simulink model "afe_inv_psm_param"  (R2026b)
settings: Solver=ode23t  StopTime=param.sim.simlength  FixedStep=tc  MaxStep=param.glb_time.tc  RelTol=1e-4
values from neighbouring files (symbols this model uses):
  param = add_template_extras(param, options)    [init_model.m]
undefined symbols (not defined in the file or in its folder): magnitude, omega_m_bez
libraries: fl_lib x330, nesl_utility x174, igbt_simple_2th_lib x12, moving_average_filter x10, moving_average_filter_cc x8, sl_discontinuities x3, single_phase_transformer_lib x3, linear_double_integrator_observer_ccaller x2, discrete_time_low_pass_filter x2, threephase_inductor_lib x2, three_phase_pwm_modulator x2, three_phase_inverter_ideal_switch_based_model x2
(part 2 of 13)

== system afe_inv_psm_param/grid/power meter iec mfunc ==
  Bus Selector : BusSelector  OutputSignals=Q1p,Q1n,P1n,P1p,U1n,U1p,i_act_1n,i_react_1n,i_act_1p,i_react_1p
  Constant : Constant  Value=param.glb_time.ts_afe
  Step : Step  Time=0.025  InitialValue=1  FinalValue=0  SampleTime=0
  To Workspace1 : ToWorkspace  VariableName=i_react_1n  SampleTime=param.glb_time.ts_afe
      settings: MaxDataPoints=param.glb_time.Ns_afe
  To Workspace2 : ToWorkspace  VariableName=i_react_1p  SampleTime=param.glb_time.ts_afe
      settings: MaxDataPoints=param.glb_time.Ns_afe
  To Workspace3 : ToWorkspace  VariableName=i_act_1n  SampleTime=param.glb_time.ts_afe
      settings: MaxDataPoints=param.glb_time.Ns_afe
  To Workspace4 : ToWorkspace  VariableName=i_act_1p  SampleTime=param.glb_time.ts_afe
      settings: MaxDataPoints=param.glb_time.Ns_afe
  To Workspace5 : ToWorkspace  VariableName=u1p  SampleTime=param.glb_time.ts_afe
      settings: MaxDataPoints=param.glb_time.Ns_afe
  To Workspace6 : ToWorkspace  VariableName=u1n  SampleTime=param.glb_time.ts_afe
      settings: MaxDataPoints=param.glb_time.Ns_afe
  Zero-Order Hold{,1..5} (6 alike) : ZeroOrderHold  SampleTime=param.glb_time.ts_afe
  three_phase_power_meter_iec : MATLAB Function  TreatAsAtomicUnit=on  SystemSampleTime=param.glb_time.ts_afe
  tag scope: P1n_global=global, P1p_global=global, Q1n_global=global, Q1p_global=global
  wires:
  Bus Selector/6 -> To Workspace5/1  "<U1p>"
  Bus Selector/8 -> To Workspace1/1  "<i_react_1n>"
  Bus Selector/10 -> To Workspace2/1  "<i_react_1p>"
  Bus Selector/5 -> To Workspace6/1  "<U1n>"
  Bus Selector/4 -> [P1p_global]  "<P1p>"
  Bus Selector/2 -> [Q1n_global]  "<Q1n>"
  Bus Selector/1 -> [Q1p_global]  "<Q1p>"
  Bus Selector/7 -> To Workspace3/1  "<i_act_1n>"
  Bus Selector/9 -> To Workspace4/1  "<i_act_1p>"
  Bus Selector/3 -> [P1n_global]  "<P1n>"
  three_phase_power_meter_iec/1(m) -> Bus Selector/1
  Zero-Order Hold/1 -> three_phase_power_meter_iec/1(phase)
  Zero-Order Hold2/1 -> three_phase_power_meter_iec/3(i_abc)
  [phase_grid_emulator] -> Zero-Order Hold/1
  Step/1 -> Zero-Order Hold5/1
  Zero-Order Hold3/1 -> three_phase_power_meter_iec/4(omega)
  Zero-Order Hold4/1 -> three_phase_power_meter_iec/5(ts)
  [ug_abc] -> Zero-Order Hold1/1
  Zero-Order Hold5/1 -> three_phase_power_meter_iec/6(enable_time)
  [ig_abc] -> Zero-Order Hold2/1
  [omega_grid_emulator] -> Zero-Order Hold3/1
  Constant/1 -> Zero-Order Hold4/1
  Zero-Order Hold1/1 -> three_phase_power_meter_iec/2(u_abc)

== system afe_inv_psm_param/grid/threephase_vi_measures ==
  Bus Creator : BusCreator  Inputs=6
  Current Sensor : fl_lib/Electrical/Electrical Sensors/Current Sensor
  Current Sensor1 : fl_lib/Electrical/Electrical Sensors/Current Sensor
  Current Sensor2 : fl_lib/Electrical/Electrical Sensors/Current Sensor
  Electrical Reference1 : fl_lib/Electrical/Electrical Elements/Electrical Reference
  Selector : Selector  InputPortWidth=6  IndexOptions=Index vector (dialog)  Indices=[1 2 3]  OutputSizes=1  RuntimeRangeChecks=off
  Selector1 : Selector  InputPortWidth=6  IndexOptions=Index vector (dialog)  Indices=[4 5 6]  OutputSizes=1  RuntimeRangeChecks=off
  Voltage Sensor : fl_lib/Electrical/Electrical Sensors/Voltage Sensor
  Voltage Sensor1 : fl_lib/Electrical/Electrical Sensors/Voltage Sensor
  Voltage Sensor2 : fl_lib/Electrical/Electrical Sensors/Voltage Sensor
  ia_grid : nesl_utility/PS-Simulink Converter  PhysicalDomain=network_engine_domain  SubClassName=ps_output  LeftPortType=input  RightPortType=output  PseudoPeriodic=off  Frequencies=[]  VectorFormat=1-D array  Unit=A  AffineConversion=off
  ib_grid : nesl_utility/PS-Simulink Converter  PhysicalDomain=network_engine_domain  SubClassName=ps_output  LeftPortType=input  RightPortType=output  PseudoPeriodic=off  Frequencies=[]  VectorFormat=1-D array  Unit=A  AffineConversion=off
  ic_grid : nesl_utility/PS-Simulink Converter  PhysicalDomain=network_engine_domain  SubClassName=ps_output  LeftPortType=input  RightPortType=output  PseudoPeriodic=off  Frequencies=[]  VectorFormat=1-D array  Unit=A  AffineConversion=off
  ig_abc/ug_abc : Scope  NumInputPorts=2
      settings: SampleTime=param.glb_time.tc  ActiveDisplayYMinimum=-728.92703752654245  ActiveDisplayYMaximum=734.90808013997  DataLoggingVariableName=ScopeData2
  ua_grid : nesl_utility/PS-Simulink Converter  PhysicalDomain=network_engine_domain  SubClassName=ps_output  LeftPortType=input  RightPortType=output  PseudoPeriodic=off  Frequencies=[]  VectorFormat=1-D array  Unit=V  AffineConversion=off
  ub_grid : nesl_utility/PS-Simulink Converter  PhysicalDomain=network_engine_domain  SubClassName=ps_output  LeftPortType=input  RightPortType=output  PseudoPeriodic=off  Frequencies=[]  VectorFormat=1-D array  Unit=V  AffineConversion=off
  uc_grid : nesl_utility/PS-Simulink Converter  PhysicalDomain=network_engine_domain  SubClassName=ps_output  LeftPortType=input  RightPortType=output  PseudoPeriodic=off  Frequencies=[]  VectorFormat=1-D array  Unit=V  AffineConversion=off
  Ua : PMIOPort  Side=Left
  ua : PMIOPort  Port=2  Side=Right
  Ub : PMIOPort  Port=3  Side=Left
  ub : PMIOPort  Port=4  Side=Right
  Uc : PMIOPort  Port=5  Side=Left
  uc : PMIOPort  Port=6  Side=Right
  tag scope: ig_abc=global, ug_abc=global
  wires:
  Bus Creator/1 -> Selector1/1, Selector/1  "vi_data"
  Selector/1 -> [ug_abc]
  ib_grid/1 -> Bus Creator/5  "ib"
  ia_grid/1 -> Bus Creator/4  "ia"
  ic_grid/1 -> Bus Creator/6  "ic"
  ua_grid/1 -> Bus Creator/1  "ua"
  ub_grid/1 -> Bus Creator/2  "ub"
  uc_grid/1 -> Bus Creator/3  "uc"
  Selector1/1 -> [ig_abc]
  [ug_abc] -> ig_abc/ug_abc/2  "ug_abc(line)"
  [ig_abc] -> ig_abc/ug_abc/1  "ig_abc(line)"
  connections:
  Current Sensor1/LConn1 -- Ub/RConn1 -- Voltage Sensor1/LConn1
  Electrical Reference1/LConn1 -- Voltage Sensor/RConn2 -- Voltage Sensor2/RConn2 -- Voltage Sensor1/RConn2
  Voltage Sensor/RConn1 -- ua_grid/LConn1
  Current Sensor/RConn2 -- ua/RConn1
  Voltage Sensor1/RConn1 -- ub_grid/LConn1
  Voltage Sensor2/LConn1 -- Current Sensor2/LConn1 -- Uc/RConn1
  Current Sensor/LConn1 -- Ua/RConn1 -- Voltage Sensor/LConn1
  Current Sensor1/RConn2 -- ub/RConn1
  Voltage Sensor2/RConn1 -- uc_grid/LConn1
  ib_grid/LConn1 -- Current Sensor1/RConn1
  ia_grid/LConn1 -- Current Sensor/RConn1
  ic_grid/LConn1 -- Current Sensor2/RConn1
  Current Sensor2/RConn2 -- uc/RConn1

== system afe_inv_psm_param/inverter_measurement_sim/igbt_power_losses ==
  To Workspace12 : ToWorkspace  VariableName=igbt_ploss_invQ1_sim  SampleTime=param.glb_time.tc
      settings: MaxDataPoints=param.glb_time.Nc
  To Workspace14 : ToWorkspace  VariableName=igbt_current_invQ1_sim  SampleTime=param.glb_time.tc
      settings: MaxDataPoints=param.glb_time.Nc
  To Workspace15 : ToWorkspace  VariableName=igbt_voltage_invQ1_sim  SampleTime=param.glb_time.tc
      settings: MaxDataPoints=param.glb_time.Nc
  To Workspace16 : ToWorkspace  VariableName=igbt_JH_temp_invQ1_sim  SampleTime=param.glb_time.tc
      settings: MaxDataPoints=param.glb_time.Nc
  To Workspace17 : ToWorkspace  VariableName=igbt_HA_temp_invQ1_sim  SampleTime=param.glb_time.tc
      settings: MaxDataPoints=param.glb_time.Nc
  To Workspace18 : ToWorkspace  VariableName=diode_ploss_invQ1_sim  SampleTime=param.glb_time.tc
      settings: MaxDataPoints=param.glb_time.Nc
  To Workspace19 : ToWorkspace  VariableName=diode_JH_temp_invQ1_sim  SampleTime=param.glb_time.tc
      settings: MaxDataPoints=param.glb_time.Nc
  To Workspace20 : ToWorkspace  VariableName=diode_HA_temp_invQ1_sim  SampleTime=param.glb_time.tc
      settings: MaxDataPoints=param.glb_time.Nc
  wires:
  [igbt_ploss_invQ1] -> To Workspace12/1  "igbt_ploss_invQ1"
  [igbt_current_invQ1] -> To Workspace14/1  "igbt_current_invQ1"
  [igbt_voltage_invQ1] -> To Workspace15/1  "igbt_voltage_invQ1"
  [diode_JH_temp_invQ1] -> To Workspace19/1  "diode_JH_temp_invQ1"
  [igbt_JH_temp_invQ1] -> To Workspace16/1  "igbt_JH_temp_invQ1"
  [diode_HA_temp_invQ1] -> To Workspace20/1  "diode_HA_temp_invQ1"
  [igbt_HA_temp_invQ1] -> To Workspace17/1  "igbt_HA_temp_invQ1"
  [diode_ploss_invQ1] -> To Workspace18/1  "diode_ploss_invQ1"

== system afe_inv_psm_param/inverter_measurement_sim/module_1 ==
  To Workspace12 : ToWorkspace  VariableName=ileg_dc_inv_sim_mod1  SampleTime=param.glb_time.tc
      settings: MaxDataPoints=param.glb_time.Nc
  To Workspace14 : ToWorkspace  VariableName=is_uvw_sim_mod1  SampleTime=param.glb_time.tc
      settings: MaxDataPoints=param.glb_time.Nc
  To Workspace15 : ToWorkspace  VariableName=us_uvw_sim_mod1  SampleTime=param.glb_time.tc
      settings: MaxDataPoints=param.glb_time.Nc
  wires:
  [us_uvw_pu_mod1] -> To Workspace15/1
  [ileg_dc_inv_mod1] -> To Workspace12/1
  [is_uvw_pu_mod1] -> To Workspace14/1

== system afe_inv_psm_param/pmsm/synchronous_motor ==
  Bus Selector : BusSelector  OutputSignals=psi_r_alpha (Vs)
  Bus Selector1 : BusSelector  OutputSignals=psi_r_alpha (Vs)
  Bus Selector10 : BusSelector  OutputSignals=uq (V)
  Bus Selector11 : BusSelector  OutputSignals=ud (V)
  Bus Selector12 : BusSelector  OutputSignals=iq (A)
  Bus Selector13 : BusSelector  OutputSignals=id (A)
  Bus Selector2 : BusSelector  OutputSignals=iu (A)
  Bus Selector3 : BusSelector  OutputSignals=iv (A)
  Bus Selector4 : BusSelector  OutputSignals=iw (A)
  Bus Selector5 : BusSelector  OutputSignals=omega_elec (rad/s)
  Bus Selector6 : BusSelector  OutputSignals=phase_elec (rad)
  Bus Selector7 : BusSelector  OutputSignals=pwr_in (kW)
  Bus Selector8 : BusSelector  OutputSignals=pwr_out (kW)
  Bus Selector9 : BusSelector  OutputSignals=torque (Nm)
  Open Circuit : fl_lib/Electrical/Electrical Elements/Open Circuit  v_specify=off  v_priority=None  v=0 V  v_nominal_specify=off  v_nominal_value=1  v_nominal_unit=V
  permanent_magnet_synchronous_machine : permanent_magnet_synchronous_machine/permanent_magnet_synchronous_machine  pp=param.psm.machine.number_poles  psi_m=param.psm.machine.psi_m  Lmu=param.psm.machine.Lmu  La=param.psm.machine.La_m  Lb=param.psm.machine.Lb_m  Rs=param.psm.machine.Rs_m  Jm=param.psm.machine.Jm_m  b_linear=param.psm.machine.load_friction_m  b_quadratic=0  h5_percent=0  h7_percent=0  psi_r_u_init=param.psm.machine.psi_m  psi_r_v_init=-param.psm.machine.psi_m/2  psi_r_w_init=-param.psm.machine.psi_m/2  omega_init=0  phase_init=0  angle_error=0
  shaft : PMIOPort  Side=Right
  u : PMIOPort  Port=2  Side=Left
  v : PMIOPort  Port=3  Side=Left
  w : PMIOPort  Port=4  Side=Left
  psi_m : PMIOPort  Port=5  Side=Left
  motor_data : Outport
  tag scope: id_psm=global, iq_psm=global, iu_psm=global, iv_psm=global, iw_psm=global, omega_elec_psm=global, psi_r_alpha_psm=global, psi_r_beta_psm=global, pwr_in_psm=global, pwr_out_psm=global, theta_elec_psm=global, torque_load_psm=global, ud_psm=global, uq_psm=global
  wires:
  permanent_magnet_synchronous_machine/1 -> Bus Selector8/1, Bus Selector10/1, Bus Selector11/1, Bus Selector12/1, Bus Selector13/1, Bus Selector9/1, Bus Selector7/1, Bus Selector6/1, Bus Selector5/1, Bus Selector4/1, Bus Selector3/1, Bus Selector2/1, Bus Selector1/1, Bus Selector/1, motor_data/1
  Bus Selector/1 -> [psi_r_alpha_psm]  "<psi_r_alpha (Vs)>"
  Bus Selector1/1 -> [psi_r_beta_psm]  "<psi_r_alpha (Vs)>"
  Bus Selector2/1 -> [iu_psm]  "<iu (A)>"
  Bus Selector3/1 -> [iv_psm]  "<iv (A)>"
  Bus Selector4/1 -> [iw_psm]  "<iw (A)>"
  Bus Selector5/1 -> [omega_elec_psm]  "<omega_elec (rad/s)>"
  Bus Selector6/1 -> [theta_elec_psm]  "<phase_elec (rad)>"
  Bus Selector7/1 -> [pwr_in_psm]  "<pwr_in (kW)>"
  Bus Selector8/1 -> [pwr_out_psm]  "<pwr_out (kW)>"
  Bus Selector9/1 -> [torque_load_psm]  "<torque (Nm)>"
  Bus Selector10/1 -> [uq_psm]  "<uq (V)>"
  Bus Selector11/1 -> [ud_psm]  "<ud (V)>"
  Bus Selector12/1 -> [iq_psm]  "<iq (A)>"
  Bus Selector13/1 -> [id_psm]  "<id (A)>"
  connections:
  permanent_magnet_synchronous_machine/RConn1 -- shaft/RConn1
  permanent_magnet_synchronous_machine/LConn1 -- u/RConn1
  permanent_magnet_synchronous_machine/LConn2 -- v/RConn1
  permanent_magnet_synchronous_machine/LConn3 -- w/RConn1
  permanent_magnet_synchronous_machine/LConn4 -- psi_m/RConn1
  permanent_magnet_synchronous_machine/LConn5 -- Open Circuit/LConn1

== system afe_inv_psm_param/scopes/cable_effects ==
  cable_effects : Scope  NumInputPorts=3
      settings: SampleTime=param.glb_time.tc  ActiveDisplayYMinimum=-7.1054273576010019E-14  ActiveDisplayYMaximum=7.1054273576010019E-14  DataLoggingVariableName=ScopeData35
  wires:
  [udc_pgnd] -> cable_effects/2
  [udc_ngnd] -> cable_effects/3
  [is_uvw_cm_mod1] -> cable_effects/1

== system afe_inv_psm_param/scopes/grid_afe_side ==
  Gain7 : Gain  Gain=param.afe.hw.ibez
  Gain8 : Gain  Gain=param.afe.hw.ubez
  Gain9 : Gain  Gain=param.afe.hw.ibez
  IEC_power_meter : Scope  NumInputPorts=4
      settings: ActiveDisplayYMinimum=-221704.59704037459  ActiveDisplayYMaximum=262876.57731367293  DataLoggingVariableName=ScopeData14
  i_line_abc/u_line_abc : Scope  NumInputPorts=2
      settings: SampleTime=param.glb_time.tc  ActiveDisplayYMinimum=-1352.5734119476883  ActiveDisplayYMaximum=1505.395019752161  DataLoggingVariableName=ScopeData20
  idc/udc : Scope  NumInputPorts=2
      settings: SampleTime=param.glb_time.tc  ActiveDisplayYMinimum=-237.45231016815259  ActiveDisplayYMaximum=320.54398715417091  DataLoggingVariableName=ScopeData23
  ig_abc/ug_abc _mod1 : Scope  NumInputPorts=2
      settings: SampleTime=param.glb_time.tc  ActiveDisplayYMinimum=-4.4957016262667837  ActiveDisplayYMaximum=4.3239423057982735  DataLoggingVariableName=ScopeData22
  is_abc/us_abc _mod1 : Scope  NumInputPorts=3
      settings: SampleTime=param.glb_time.tc  ActiveDisplayYMinimum=-2620.8441075302808  ActiveDisplayYMaximum=2310.3545900694107  DataLoggingVariableName=ScopeData21
  udc voltages : Scope  NumInputPorts=2
      settings: SampleTime=param.glb_time.tc  ActiveDisplayYMinimum=-0.1691941690232826  ActiveDisplayYMaximum=1.5064339432334795  DataLoggingVariableName=ScopeData24
  wires:
  [udc_mod1] -> idc/udc/2  "udc_dclink_mod1"
  [ug_abc_pu_mod1] -> ig_abc/ug_abc _mod1/2  "ug_abc_mod1"
  Gain8/1 -> is_abc/us_abc _mod1/2  "vs_abc_mod1"
  [ic_dclink_mod1] -> idc/udc/1  "ic_dclink_mod1"
  [is_abc_pu_mod1] -> Gain7/1
  [Q1p_global] -> IEC_power_meter/2  "Q1p_global"
  [all_voltages_about_dclink] -> udc voltages/2  "all_voltages_about_dclink"
  Gain7/1 -> is_abc/us_abc _mod1/1  "is_abc_mod1"
  [iz_afe_pu_mod1] -> Gain9/1
  [i_abc_line] -> i_line_abc/u_line_abc/1  "i_abc_line"
  [u_abc_line] -> i_line_abc/u_line_abc/2  "u_abc_line"
  [P1n_global] -> IEC_power_meter/4  "P1n_global"
  [ig_abc_pu_mod1] -> ig_abc/ug_abc _mod1/1  "ig_abc_mod1"
  [vs_abc_pu_mod1] -> Gain8/1
  [vdc_pu_afe_mod1] -> udc voltages/1  "udc"
  Gain9/1 -> is_abc/us_abc _mod1/3  "iz_afe_mod1"
  [Q1n_global] -> IEC_power_meter/1  "Q1n_global"
  [P1p_global] -> IEC_power_meter/3  "P1p_global"

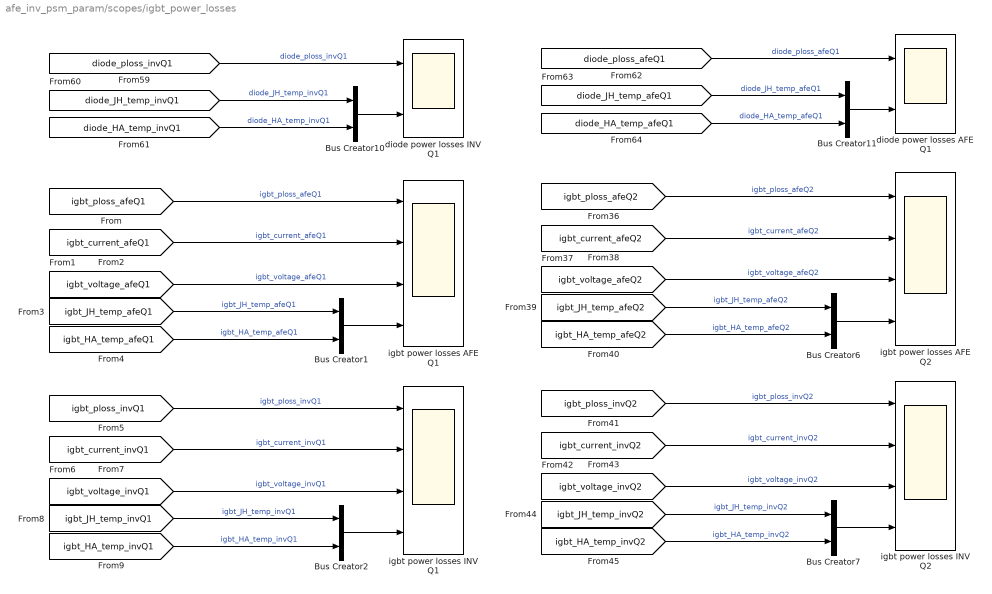
== system afe_inv_psm_param/scopes/igbt_power_losses ==
  Bus Creator{1..2,6..7,10..11} (6 alike) : BusCreator  Inputs=2
  diode power losses AFE Q1 : Scope  NumInputPorts=2
      settings: SampleTime=param.glb_time.tc  ActiveDisplayYMinimum=-0.87039317174009745  ActiveDisplayYMaximum=7.8312553964690395  DataLoggingVariableName=ScopeData32
  diode power losses INV Q1 : Scope  NumInputPorts=2
      settings: SampleTime=param.glb_time.tc  ActiveDisplayYMinimum=-1  ActiveDisplayYMaximum=1  DataLoggingVariableName=ScopeData31
  igbt power losses AFE Q1 : Scope  NumInputPorts=4
      settings: SampleTime=param.glb_time.tc  ActiveDisplayYMinimum=-49.038943467813  ActiveDisplayYMaximum=441.3504912103171  DataLoggingVariableName=ScopeData15
  igbt power losses AFE Q2 : Scope  NumInputPorts=4
      settings: SampleTime=param.glb_time.tc  ActiveDisplayYMinimum=-40.410135398015626  ActiveDisplayYMaximum=363.69121858214072  DataLoggingVariableName=ScopeData26
  igbt power losses INV Q1 : Scope  NumInputPorts=4
      settings: SampleTime=param.glb_time.tc  ActiveDisplayYMinimum=-36.37444736851036  ActiveDisplayYMaximum=327.37002631659328  DataLoggingVariableName=ScopeData16
  igbt power losses INV Q2 : Scope  NumInputPorts=4
      settings: SampleTime=param.glb_time.tc  ActiveDisplayYMinimum=-6409.6577502266955  ActiveDisplayYMaximum=762.94403267363941  DataLoggingVariableName=ScopeData27
  wires:
  [igbt_ploss_afeQ1] -> igbt power losses AFE Q1/1  "igbt_ploss_afeQ1"
  [igbt_JH_temp_invQ1] -> Bus Creator2/1  "igbt_JH_temp_invQ1"
  [diode_JH_temp_invQ1] -> Bus Creator10/1  "diode_JH_temp_invQ1"
  [igbt_HA_temp_invQ2] -> Bus Creator7/2  "igbt_HA_temp_invQ2"
  [igbt_current_afeQ2] -> igbt power losses AFE Q2/2  "igbt_current_afeQ2"
  [igbt_ploss_afeQ2] -> igbt power losses AFE Q2/1  "igbt_ploss_afeQ2"
  [igbt_current_invQ1] -> igbt power losses INV Q1/2  "igbt_current_invQ1"
  [igbt_JH_temp_afeQ1] -> Bus Creator1/1  "igbt_JH_temp_afeQ1"
  [igbt_current_invQ2] -> igbt power losses INV Q2/2  "igbt_current_invQ2"
  [diode_JH_temp_afeQ1] -> Bus Creator11/1  "diode_JH_temp_afeQ1"
  [igbt_HA_temp_invQ1] -> Bus Creator2/2  "igbt_HA_temp_invQ1"
  [igbt_JH_temp_afeQ2] -> Bus Creator6/1  "igbt_JH_temp_afeQ2"
  Bus Creator11/1 -> diode power losses AFE Q1/2
  [diode_ploss_invQ1] -> diode power losses INV Q1/1  "diode_ploss_invQ1"
  [igbt_ploss_invQ1] -> igbt power losses INV Q1/1  "igbt_ploss_invQ1"
  [igbt_HA_temp_afeQ2] -> Bus Creator6/2  "igbt_HA_temp_afeQ2"
  Bus Creator7/1 -> igbt power losses INV Q2/4
  [igbt_voltage_invQ2] -> igbt power losses INV Q2/3  "igbt_voltage_invQ2"
  Bus Creator10/1 -> diode power losses INV Q1/2
  [igbt_JH_temp_invQ2] -> Bus Creator7/1  "igbt_JH_temp_invQ2"
  [diode_HA_temp_afeQ1] -> Bus Creator11/2  "diode_HA_temp_afeQ1"
  Bus Creator1/1 -> igbt power losses AFE Q1/4
  Bus Creator6/1 -> igbt power losses AFE Q2/4
  [igbt_voltage_afeQ1] -> igbt power losses AFE Q1/3  "igbt_voltage_afeQ1"
  [igbt_current_afeQ1] -> igbt power losses AFE Q1/2  "igbt_current_afeQ1"
  [igbt_HA_temp_afeQ1] -> Bus Creator1/2  "igbt_HA_temp_afeQ1"
  [diode_ploss_afeQ1] -> diode power losses AFE Q1/1  "diode_ploss_afeQ1"
  Bus Creator2/1 -> igbt power losses INV Q1/4
  [diode_HA_temp_invQ1] -> Bus Creator10/2  "diode_HA_temp_invQ1"
  [igbt_voltage_invQ1] -> igbt power losses INV Q1/3  "igbt_voltage_invQ1"
  [igbt_ploss_invQ2] -> igbt power losses INV Q2/1  "igbt_ploss_invQ2"
  [igbt_voltage_afeQ2] -> igbt power losses AFE Q2/3  "igbt_voltage_afeQ2"

== system afe_inv_psm_param/scopes/machine_side ==
  Bus Creator3 : BusCreator  Inputs=2
  Bus Creator4 : BusCreator  Inputs=2
  Bus Creator5 : BusCreator  Inputs=2
  From56 : From  Commented=on  GotoTag=inverter_voltage_ee_phase_u
  From57 : From  Commented=on  GotoTag=inverter_voltage_ee_phase_v
  From58 : From  Commented=on  GotoTag=inverter_voltage_ee_phase_w
  Gain1 : Gain  Gain=1e-3
  LTI System : cstblocks_lti/LTI System  sys=param.ctrl.filters.inv.SOF_50Hz.ss_c  IC=[]  PadeOrder=0
  LTI System1 : cstblocks_lti/LTI System  sys=param.ctrl.filters.inv.SOF_50Hz.ss_c  IC=[]  PadeOrder=0
  inverter_voltage_ee : Scope  Commented=on  NumInputPorts=3
      settings: SampleTime=param.sim.tc  ActiveDisplayYMinimum=-207.5782073641667  ActiveDisplayYMaximum=1301.7632755987056  DataLoggingVariableName=ScopeData30
  is_uvw/us_uvw : Scope  NumInputPorts=2
      settings: SampleTime=param.glb_time.tc  ActiveDisplayYMinimum=-1.2325569675038333  ActiveDisplayYMaximum=1.2339333833020862  DataLoggingVariableName=ScopeData25
  motor currents : Scope  NumInputPorts=3
      settings: SampleTime=param.glb_time.tc  ActiveDisplayYMinimum=-232.58671124644178  ActiveDisplayYMaximum=232.76282128626991  DataLoggingVariableName=ScopeData17
  motor dq : Scope  NumInputPorts=2
      settings: SampleTime=param.glb_time.tc  ActiveDisplayYMinimum=-850.02239826316088  ActiveDisplayYMaximum=207.16586596148719  DataLoggingVariableName=ScopeData18
  motor mech : Scope  NumInputPorts=3
      settings: SampleTime=param.glb_time.tc  ActiveDisplayYMinimum=-2.216582738378952  ActiveDisplayYMaximum=19.949244645410573  DataLoggingVariableName=ScopeData11
  phi_alpha_pmsm/phi_beta_pmsm : Scope  NumInputPorts=2
      settings: SampleTime=param.glb_time.tc  ActiveDisplayYMinimum=-4.8008048511588592  ActiveDisplayYMaximum=4.8008564448893649  DataLoggingVariableName=ScopeData19
  wires:
  [iu_psm] -> motor currents/1  "iu_psm"
  [psi_r_beta_psm] -> phi_alpha_pmsm/phi_beta_pmsm/2
  [id_psm] -> Bus Creator4/2  "id_psm"
  [ud_psm] -> Bus Creator3/1  "ud_psm"
  Bus Creator4/1 -> motor dq/2
  [iq_psm] -> Bus Creator4/1  "iq_psm"
  [uq_psm] -> Bus Creator3/2  "uq_psm"
  Bus Creator3/1 -> motor dq/1
  [psi_r_alpha_psm] -> phi_alpha_pmsm/phi_beta_pmsm/1
  [iv_psm] -> motor currents/2  "iv_psm"
  [iw_psm] -> motor currents/3  "iw_psm"
  [pwr_in_psm] -> LTI System/1
  LTI System1/1 -> Bus Creator5/2  "pwr_out_psm (kW)"
  [torque_load_psm] -> Gain1/1
  LTI System/1 -> Bus Creator5/1  "pin_psm (kW)"
  Gain1/1 -> motor mech/2  "torque_load_psm (kNm)"
  [rpm_motor] -> motor mech/1  "omega_elec_psm (rpm)"
  Bus Creator5/1 -> motor mech/3
  [pwr_out_psm] -> LTI System1/1
  [us_uvw_pu_mod1] -> is_uvw/us_uvw/2  "us_uvw_pu_mod1"
  [is_uvw_pu_mod1] -> is_uvw/us_uvw/1  "is_uvw_pu_mod1"
  From58/1 -> inverter_voltage_ee/3  "inverter_voltage_ee_phase_w"
  From56/1 -> inverter_voltage_ee/1  "inverter_voltage_ee_phase_u"
  From57/1 -> inverter_voltage_ee/2  "inverter_voltage_ee_phase_v"

== system afe_inv_psm_param/scopes/mosfet_power_losses ==
  Bus Creator8 : BusCreator  Inputs=2
  Bus Creator9 : BusCreator  Inputs=2
  mosfet power losses INV Q1 : Scope  NumInputPorts=4
      settings: SampleTime=param.glb_time.tc  ActiveDisplayYMinimum=-52.647210306071649  ActiveDisplayYMaximum=473.81757031333393  DataLoggingVariableName=ScopeData28
  mosfet power losses INV Q2 : Scope  NumInputPorts=4
      settings: SampleTime=param.glb_time.tc  ActiveDisplayYMinimum=-60.051099059926763  ActiveDisplayYMaximum=540.45256909803  DataLoggingVariableName=ScopeData29
  wires:
  [mosfet_current_invQ2] -> mosfet power losses INV Q2/3  "mosfet_current_invQ2"
  [mosfet_voltage_invQ1] -> mosfet power losses INV Q1/2  "mosfet_voltage_invQ1"
  [mosfet_HA_temp_invQ2] -> Bus Creator9/2  "mosfet_HA_temp_invQ2"
  [mosfet_JH_temp_invQ2] -> Bus Creator9/1  "mosfet_JH_temp_invQ2"
  [mosfet_ploss_invQ1] -> mosfet power losses INV Q1/1  "mosfet_ploss_invQ1"
  [mosfet_HA_temp_invQ1] -> Bus Creator8/2  "mosfet_HA_temp_invQ1"
  [mosfet_current_invQ1] -> mosfet power losses INV Q1/3  "mosfet_current_invQ1"
  Bus Creator8/1 -> mosfet power losses INV Q1/4
  [mosfet_voltage_invQ2] -> mosfet power losses INV Q2/2  "mosfet_voltage_invQ2"
  [mosfet_ploss_invQ2] -> mosfet power losses INV Q2/1  "mosfet_ploss_invQ2"
  Bus Creator9/1 -> mosfet power losses INV Q2/4
  [mosfet_JH_temp_invQ1] -> Bus Creator8/1  "mosfet_JH_temp_invQ1"

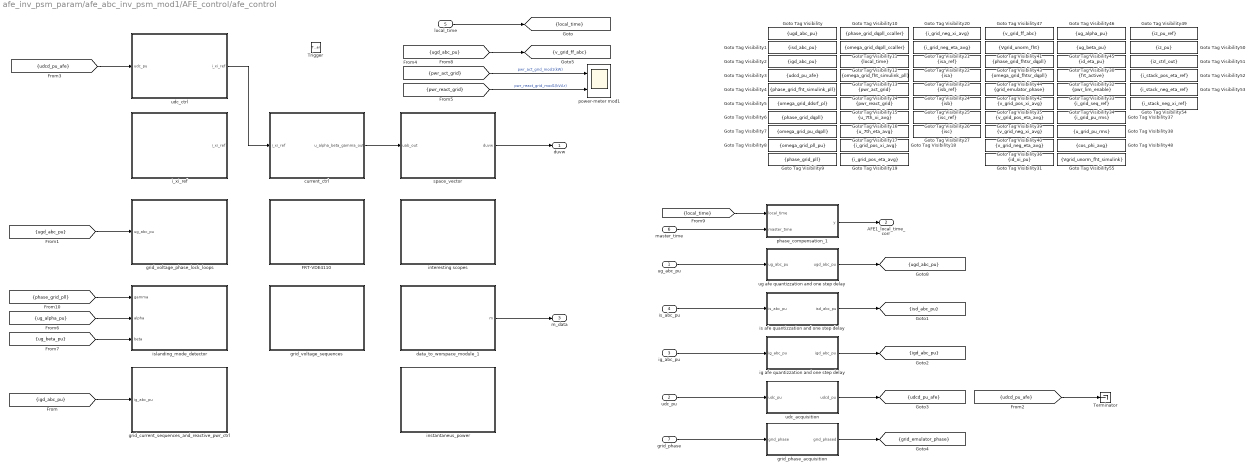
== system afe_inv_psm_param/afe_abc_inv_psm_mod1/AFE_control/afe_control ==
  ug_abc_pu : Inport
  udc_pu : Inport  Port=2
  ig_abc_pu : Inport  Port=3
  is_abc_pu : Inport  Port=4
  local_time : Inport  Port=5
  master_time : Inport  Port=6
  grid_phase : Inport  Port=7
  Trigger : TriggerPort  VariantControl=(inherit)  PortDimensions=1
  FRT-VDE4110 : Subsystem
  Goto Tag Visibility : GotoTagVisibility  GotoTag=ugd_abc_pu
  Goto Tag Visibility1 : GotoTagVisibility  GotoTag=isd_abc_pu
  Goto Tag Visibility10 : GotoTagVisibility  GotoTag=phase_grid_dqpll_ccaller
  Goto Tag Visibility11 : GotoTagVisibility  GotoTag=omega_grid_dqpll_ccaller
  Goto Tag Visibility12 : GotoTagVisibility  GotoTag=local_time
  Goto Tag Visibility13 : GotoTagVisibility  GotoTag=omega_grid_fht_simulink_pll
  Goto Tag Visibility14 : GotoTagVisibility  GotoTag=pwr_act_grid
  Goto Tag Visibility15 : GotoTagVisibility  GotoTag=pwr_react_grid
  Goto Tag Visibility16 : GotoTagVisibility  GotoTag=u_7th_xi_avg
  Goto Tag Visibility17 : GotoTagVisibility  GotoTag=u_7th_eta_avg
  Goto Tag Visibility18 : GotoTagVisibility  GotoTag=i_grid_pos_xi_avg
  Goto Tag Visibility19 : GotoTagVisibility  GotoTag=i_grid_pos_eta_avg
  Goto Tag Visibility2 : GotoTagVisibility  GotoTag=igd_abc_pu
  Goto Tag Visibility20 : GotoTagVisibility  GotoTag=i_grid_neg_xi_avg
  Goto Tag Visibility21 : GotoTagVisibility  GotoTag=i_grid_neg_eta_avg
  Goto Tag Visibility22 : GotoTagVisibility  GotoTag=isa_ref
  Goto Tag Visibility23 : GotoTagVisibility  GotoTag=isa
  Goto Tag Visibility24 : GotoTagVisibility  GotoTag=isb_ref
  Goto Tag Visibility25 : GotoTagVisibility  GotoTag=isb
  Goto Tag Visibility26 : GotoTagVisibility  GotoTag=isc_ref
  Goto Tag Visibility27 : GotoTagVisibility  GotoTag=isc
  Goto Tag Visibility3 : GotoTagVisibility  GotoTag=udcd_pu_afe
  Goto Tag Visibility30 : GotoTagVisibility  GotoTag=id_eta_pu
  Goto Tag Visibility31 : GotoTagVisibility  GotoTag=id_xi_pu
  Goto Tag Visibility32 : GotoTagVisibility  GotoTag=frt_active
  Goto Tag Visibility33 : GotoTagVisibility  GotoTag=pwr_lim_enable
  Goto Tag Visibility34 : GotoTagVisibility  GotoTag=i_grid_seq_ref
  Goto Tag Visibility35 : GotoTagVisibility  GotoTag=v_grid_pos_xi_avg
  Goto Tag Visibility36 : GotoTagVisibility  GotoTag=v_grid_neg_eta_avg
  Goto Tag Visibility37 : GotoTagVisibility  GotoTag=i_grid_pu_rms
  Goto Tag Visibility38 : GotoTagVisibility  GotoTag=u_grid_pu_rms
  Goto Tag Visibility39 : GotoTagVisibility  GotoTag=v_grid_pos_eta_avg
  Goto Tag Visibility4 : GotoTagVisibility  GotoTag=phase_grid_fht_simulink_pll
  Goto Tag Visibility40 : GotoTagVisibility  GotoTag=v_grid_neg_xi_avg
  Goto Tag Visibility41 : GotoTagVisibility  GotoTag=Vgrid_unorm_fht
  Goto Tag Visibility42 : GotoTagVisibility  GotoTag=grid_emulator_phase
  Goto Tag Visibility43 : GotoTagVisibility  GotoTag=phase_grid_fhtsr_dqpll
  Goto Tag Visibility44 : GotoTagVisibility  GotoTag=omega_grid_fhtsr_dqpll
  Goto Tag Visibility45 : GotoTagVisibility  GotoTag=ug_beta_pu
  Goto Tag Visibility46 : GotoTagVisibility  GotoTag=ug_alpha_pu
  Goto Tag Visibility47 : GotoTagVisibility  GotoTag=v_grid_ff_abc
  Goto Tag Visibility48 : GotoTagVisibility  GotoTag=cos_phi_avg
  Goto Tag Visibility49 : GotoTagVisibility  GotoTag=iz_pu_ref
  Goto Tag Visibility5 : GotoTagVisibility  GotoTag=omega_grid_ddsrf_pl
  Goto Tag Visibility50 : GotoTagVisibility  GotoTag=iz_pu
  Goto Tag Visibility51 : GotoTagVisibility  GotoTag=iz_ctrl_out
  Goto Tag Visibility52 : GotoTagVisibility  GotoTag=i_stack_pos_eta_ref
  Goto Tag Visibility53 : GotoTagVisibility  GotoTag=i_stack_neg_eta_ref
  Goto Tag Visibility54 : GotoTagVisibility  GotoTag=i_stack_neg_xi_ref
  Goto Tag Visibility55 : GotoTagVisibility  GotoTag=Vgrid_unorm_fht_simulink
  Goto Tag Visibility6 : GotoTagVisibility  GotoTag=phase_grid_dqpll
  Goto Tag Visibility7 : GotoTagVisibility  GotoTag=omega_grid_pu_dqpll
  Goto Tag Visibility8 : GotoTagVisibility  GotoTag=omega_grid_pll_pu
  Goto Tag Visibility9 : GotoTagVisibility  GotoTag=phase_grid_pll
  Terminator : Terminator
  current_ctrl : Subsystem
  data_to_worspace_module_1 : Subsystem
  grid_current_sequences_and_reactive_pwr_ctrl : Subsystem
  grid_phase_acquisition : Subsystem
  grid_voltage_phase_lock_loops : Subsystem
  grid_voltage_sequences : Subsystem
  i_xi_ref : Subsystem
  ig afe quantizzation and one step delay : Subsystem
  instantaneus_power : Subsystem
  interesting scopes : Subsystem
  is afe quantizzation and one step delay : Subsystem
  islanding_mode_detector : Subsystem
  phase_compensation_1 : Subsystem
  power-meter mod1 : Scope  NumInputPorts=2
      settings: ActiveDisplayYMinimum=-67.030069207436668  ActiveDisplayYMaximum=116.57466656594397  DataLoggingVariableName=ScopeData9
  space_vector : Subsystem
  udc_acquisition : Subsystem
  udc_ctrl : Subsystem
  ug afe quantizzation and one step delay : Subsystem
  duvw : Outport
  AFE1_local_time_corr : Outport  Port=2
  m_data : Outport  Port=3
  tag scope: grid_emulator_phase=scoped, igd_abc_pu=scoped, isd_abc_pu=scoped, local_time=scoped, udcd_pu_afe=scoped, ugd_abc_pu=scoped, v_grid_ff_abc=scoped
  wires:
  ug_abc_pu/1 -> ug afe quantizzation and one step delay/1(ug_abc_pu)
  current_ctrl/1(u_alpha_beta_gamma_out) -> space_vector/1(uab_out)
  space_vector/1(duvw) -> duvw/1
  is_abc_pu/1 -> is afe quantizzation and one step delay/1(is_abc_pu)
  ig_abc_pu/1 -> ig afe quantizzation and one step delay/1(ig_abc_pu)
  [ugd_abc_pu] -> grid_voltage_phase_lock_loops/1(ug_abc_pu)
  [igd_abc_pu] -> grid_current_sequences_and_reactive_pwr_ctrl/1(ig_abc_pu)
  [udcd_pu_afe] -> udc_ctrl/1(udc_pu)
  udc_pu/1 -> udc_acquisition/1(udc_pu)
  udc_acquisition/1(udcd_pu) -> [udcd_pu_afe]
  [pwr_react_grid] -> power-meter mod1/2  "pwr_react_grid_mod1(kVAr)"
  [pwr_act_grid] -> power-meter mod1/1  "pwr_act_grid_mod1(kW)"
  [phase_grid_pll] -> islanding_mode_detector/1(gamma)
  [ug_alpha_pu] -> islanding_mode_detector/2(alpha)
  ug afe quantizzation and one step delay/1(ugd_abc_pu) -> [ugd_abc_pu]
  is afe quantizzation and one step delay/1(isd_abc_pu) -> [isd_abc_pu]
  ig afe quantizzation and one step delay/1(igd_abc_pu) -> [igd_abc_pu]
  [ug_beta_pu] -> islanding_mode_detector/3(beta)
  local_time/1 -> [local_time]
  master_time/1 -> phase_compensation_1/2(master_time)
  phase_compensation_1/1(y) -> AFE1_local_time_corr/1
  [local_time] -> phase_compensation_1/1(local_time)
  grid_phase/1 -> grid_phase_acquisition/1(grid_phase)
  grid_phase_acquisition/1(grid_phased) -> [grid_emulator_phase]
  [ugd_abc_pu] -> [v_grid_ff_abc]
  data_to_worspace_module_1/1(m) -> m_data/1
  [udcd_pu_afe] -> Terminator/1
  udc_ctrl/1(i_xi_ref) -> current_ctrl/1(i_xi_ref)

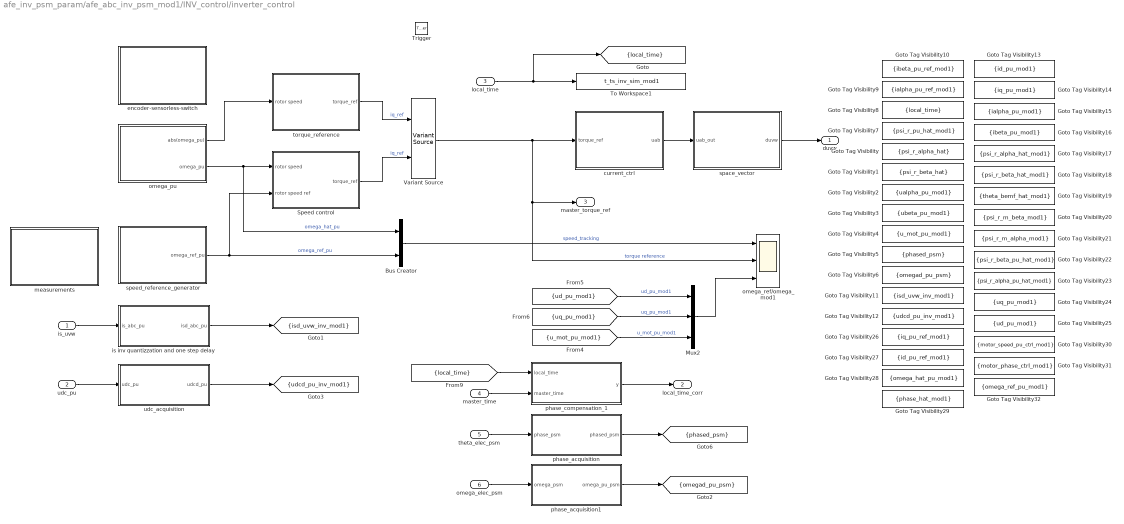
== system afe_inv_psm_param/afe_abc_inv_psm_mod1/INV_control/inverter_control ==
  is_uvw : Inport
  udc_pu : Inport  Port=2
  local_time : Inport  Port=3
  master_time : Inport  Port=4
  theta_elec_psm : Inport  Port=5
  omega_elec_psm : Inport  Port=6
  Trigger : TriggerPort  VariantControl=(inherit)  PortDimensions=1
  Bus Creator : BusCreator  Inputs=2
  Goto Tag Visibility : GotoTagVisibility  GotoTag=psi_r_alpha_hat
  Goto Tag Visibility1 : GotoTagVisibility  GotoTag=psi_r_beta_hat
  Goto Tag Visibility10 : GotoTagVisibility  GotoTag=ibeta_pu_ref_mod1
  Goto Tag Visibility11 : GotoTagVisibility  GotoTag=isd_uvw_inv_mod1
  Goto Tag Visibility12 : GotoTagVisibility  GotoTag=udcd_pu_inv_mod1
  Goto Tag Visibility13 : GotoTagVisibility  GotoTag=id_pu_mod1
  Goto Tag Visibility14 : GotoTagVisibility  GotoTag=iq_pu_mod1
  Goto Tag Visibility15 : GotoTagVisibility  GotoTag=ialpha_pu_mod1
  Goto Tag Visibility16 : GotoTagVisibility  GotoTag=ibeta_pu_mod1
  Goto Tag Visibility17 : GotoTagVisibility  GotoTag=psi_r_alpha_hat_mod1
  Goto Tag Visibility18 : GotoTagVisibility  GotoTag=psi_r_beta_hat_mod1
  Goto Tag Visibility19 : GotoTagVisibility  GotoTag=theta_bemf_hat_mod1
  Goto Tag Visibility2 : GotoTagVisibility  GotoTag=ualpha_pu_mod1
  Goto Tag Visibility20 : GotoTagVisibility  GotoTag=psi_r_m_beta_mod1
  Goto Tag Visibility21 : GotoTagVisibility  GotoTag=psi_r_m_alpha_mod1
  Goto Tag Visibility22 : GotoTagVisibility  GotoTag=psi_r_beta_pu_hat_mod1
  Goto Tag Visibility23 : GotoTagVisibility  GotoTag=psi_r_alpha_pu_hat_mod1
  Goto Tag Visibility24 : GotoTagVisibility  GotoTag=uq_pu_mod1
  Goto Tag Visibility25 : GotoTagVisibility  GotoTag=ud_pu_mod1
  Goto Tag Visibility26 : GotoTagVisibility  GotoTag=iq_pu_ref_mod1
  Goto Tag Visibility27 : GotoTagVisibility  GotoTag=id_pu_ref_mod1
  Goto Tag Visibility28 : GotoTagVisibility  GotoTag=omega_hat_pu_mod1
  Goto Tag Visibility29 : GotoTagVisibility  GotoTag=phase_hat_mod1
  Goto Tag Visibility3 : GotoTagVisibility  GotoTag=ubeta_pu_mod1
  Goto Tag Visibility30 : GotoTagVisibility  GotoTag=motor_speed_pu_ctrl_mod1
  Goto Tag Visibility31 : GotoTagVisibility  GotoTag=motor_phase_ctrl_mod1
  Goto Tag Visibility32 : GotoTagVisibility  GotoTag=omega_ref_pu_mod1
  Goto Tag Visibility4 : GotoTagVisibility  GotoTag=u_mot_pu_mod1
  Goto Tag Visibility5 : GotoTagVisibility  GotoTag=phased_psm
  Goto Tag Visibility6 : GotoTagVisibility  GotoTag=omegad_pu_psm
  Goto Tag Visibility7 : GotoTagVisibility  GotoTag=psi_r_pu_hat_mod1
  Goto Tag Visibility8 : GotoTagVisibility  GotoTag=local_time
  Goto Tag Visibility9 : GotoTagVisibility  GotoTag=ialpha_pu_ref_mod1
  Mux2 : Mux  Inputs=3
  Speed control : Subsystem
  To Workspace1 : ToWorkspace  VariableName=t_ts_inv_sim_mod1  SampleTime=-1
      settings: MaxDataPoints=param.glb_time.Ns_afe
  Variant Source : VariantSource  VariantControls={param.psm.mode.use_torque_curve == 1, param.psm.mode.use_speed_control == 1}
  current_ctrl : Subsystem
  encoder-sensorless-switch : Subsystem
  is inv quantizzation and one step delay : Subsystem
  measurements : Subsystem
  omega_pu : Subsystem
  omega_ref/omega_mod1 : Scope  NumInputPorts=3
      settings: ActiveDisplayYMinimum=-0.50152951780340871  ActiveDisplayYMaximum=1.1460012033149098  DataLoggingVariableName=ScopeData3
  phase_acquisition : Subsystem
  phase_acquisition1 : Subsystem
  phase_compensation_1 : Subsystem
  space_vector : Subsystem
  speed_reference_generator : Subsystem
  torque_reference : Subsystem
  udc_acquisition : Subsystem
  duvw : Outport  VectorParamsAs1DForOutWhenUnconnected=off
  local_time_corr : Outport  Port=2
  master_torque_ref : Outport  Port=3  VectorParamsAs1DForOutWhenUnconnected=off
  tag scope: isd_uvw_inv_mod1=scoped, local_time=scoped, omegad_pu_psm=scoped, phased_psm=scoped, udcd_pu_inv_mod1=scoped
  wires:
  speed_reference_generator/1(omega_ref_pu) -> Speed control/2(rotor speed ref), Bus Creator/2  "omega_ref_pu"
  Bus Creator/1 -> omega_ref/omega_mod1/1  "speed_tracking"
  Variant Source/1 -> current_ctrl/1(torque_ref), master_torque_ref/1, omega_ref/omega_mod1/2  "torque reference"
  [ud_pu_mod1] -> Mux2/1  "ud_pu_mod1"
  [uq_pu_mod1] -> Mux2/2  "uq_pu_mod1"
  Mux2/1 -> omega_ref/omega_mod1/3
  [u_mot_pu_mod1] -> Mux2/3  "u_mot_pu_mod1"
  omega_pu/2(omega_pu) -> Bus Creator/1, Speed control/1(rotor speed)  "omega_hat_pu"
  omega_pu/1(abs(omega_pu)) -> torque_reference/1(rotor speed)
  torque_reference/1(torque_ref) -> Variant Source/1  "iq_ref"
  Speed control/1(torque_ref) -> Variant Source/2  "iq_ref"
  udc_acquisition/1(udcd_pu) -> [udcd_pu_inv_mod1]
  udc_pu/1 -> udc_acquisition/1(udc_pu)
  is_uvw/1 -> is inv quantizzation and one step delay/1(is_abc_pu)
  is inv quantizzation and one step delay/1(isd_abc_pu) -> [isd_uvw_inv_mod1]
  local_time/1 -> To Workspace1/1, [local_time]
  current_ctrl/1(uab) -> space_vector/1(uab_out)
  space_vector/1(duvw) -> duvw/1
  master_time/1 -> phase_compensation_1/2(master_time)
  [local_time] -> phase_compensation_1/1(local_time)
  phase_compensation_1/1(y) -> local_time_corr/1
  phase_acquisition/1(phased_psm) -> [phased_psm]
  theta_elec_psm/1 -> phase_acquisition/1(phase_psm)
  omega_elec_psm/1 -> phase_acquisition1/1(omega_psm)
  phase_acquisition1/1(omega_pu_psm) -> [omegad_pu_psm]

== system afe_inv_psm_param/afe_abc_inv_psm_mod1/LCL_filter/threephase_vi_measures_stack ==
  Bus Creator : BusCreator  Inputs=6
  Current Sensor : fl_lib/Electrical/Electrical Sensors/Current Sensor
  Current Sensor1 : fl_lib/Electrical/Electrical Sensors/Current Sensor
  Current Sensor2 : fl_lib/Electrical/Electrical Sensors/Current Sensor
  Electrical Reference1 : fl_lib/Electrical/Electrical Elements/Electrical Reference
  Gain : Gain  Gain=1/3
  Gain1 : Gain  Gain=1/param.afe.hw.ubez
  Gain2 : Gain  Gain=1/param.afe.hw.ubez
  Gain3 : Gain  Gain=1/param.afe.hw.ubez
  Gain4 : Gain  Gain=1/param.afe.hw.ibez
  Gain5 : Gain  Gain=1/param.afe.hw.ibez
  Gain6 : Gain  Gain=1/param.afe.hw.ibez
  Selector : Selector  InputPortWidth=6  IndexOptions=Index vector (dialog)  Indices=[1 2 3]  OutputSizes=1  RuntimeRangeChecks=off
  Selector1 : Selector  InputPortWidth=6  IndexOptions=Index vector (dialog)  Indices=[4 5 6]  OutputSizes=1  RuntimeRangeChecks=off
  Sum : Sum  Inputs=+++
  Voltage Sensor : fl_lib/Electrical/Electrical Sensors/Voltage Sensor
  Voltage Sensor1 : fl_lib/Electrical/Electrical Sensors/Voltage Sensor
  Voltage Sensor2 : fl_lib/Electrical/Electrical Sensors/Voltage Sensor
  ia_afe : nesl_utility/PS-Simulink Converter  PhysicalDomain=network_engine_domain  SubClassName=ps_output  LeftPortType=input  RightPortType=output  PseudoPeriodic=off  Frequencies=[]  VectorFormat=1-D array  Unit=A  AffineConversion=off
  ib_afe : nesl_utility/PS-Simulink Converter  PhysicalDomain=network_engine_domain  SubClassName=ps_output  LeftPortType=input  RightPortType=output  PseudoPeriodic=off  Frequencies=[]  VectorFormat=1-D array  Unit=A  AffineConversion=off
  ic_afe : nesl_utility/PS-Simulink Converter  PhysicalDomain=network_engine_domain  SubClassName=ps_output  LeftPortType=input  RightPortType=output  PseudoPeriodic=off  Frequencies=[]  VectorFormat=1-D array  Unit=A  AffineConversion=off
  ua_afe : nesl_utility/PS-Simulink Converter  PhysicalDomain=network_engine_domain  SubClassName=ps_output  LeftPortType=input  RightPortType=output  PseudoPeriodic=off  Frequencies=[]  VectorFormat=1-D array  Unit=V  AffineConversion=off
  ub_afe : nesl_utility/PS-Simulink Converter  PhysicalDomain=network_engine_domain  SubClassName=ps_output  LeftPortType=input  RightPortType=output  PseudoPeriodic=off  Frequencies=[]  VectorFormat=1-D array  Unit=V  AffineConversion=off
  uc_afe : nesl_utility/PS-Simulink Converter  PhysicalDomain=network_engine_domain  SubClassName=ps_output  LeftPortType=input  RightPortType=output  PseudoPeriodic=off  Frequencies=[]  VectorFormat=1-D array  Unit=V  AffineConversion=off
  Ua : PMIOPort  Side=Left
  ua : PMIOPort  Port=2  Side=Right
  Ub : PMIOPort  Port=3  Side=Left
  ub : PMIOPort  Port=4  Side=Right
  Uc : PMIOPort  Port=5  Side=Left
  uc : PMIOPort  Port=6  Side=Right
  tag scope: is_abc_pu_mod1=global, iz_afe_pu_mod1=global, vs_abc_pu_mod1=global
  wires:
  Bus Creator/1 -> Selector/1, Selector1/1  "vi_data"
  Selector/1 -> [vs_abc_pu_mod1]
  ib_afe/1 -> Gain4/1  "ib_afe"
  ia_afe/1 -> Gain6/1  "ia_afe"
  ic_afe/1 -> Gain5/1  "ic_afe"
  ua_afe/1 -> Gain1/1  "ua_afe"
  ub_afe/1 -> Gain2/1  "ub_afe"
  uc_afe/1 -> Gain3/1  "uc_afe"
  Selector1/1 -> [is_abc_pu_mod1]
  Sum/1 -> Gain/1
  Gain/1 -> [iz_afe_pu_mod1]
  Gain1/1 -> Bus Creator/1  "ua_afe_pu"
  Gain2/1 -> Bus Creator/2  "ub_afe_pu"
  Gain3/1 -> Bus Creator/3  "uc_afe_pu"
  Gain6/1 -> Sum/1, Bus Creator/4  "ia_afe_pu"
  Gain4/1 -> Sum/2, Bus Creator/5  "ib_afe_pu"
  Gain5/1 -> Bus Creator/6, Sum/3  "ic_afe_pu"
  connections:
  Current Sensor1/LConn1 -- Ub/RConn1 -- Voltage Sensor1/LConn1
  Electrical Reference1/LConn1 -- Voltage Sensor/RConn2 -- Voltage Sensor2/RConn2 -- Voltage Sensor1/RConn2
  Voltage Sensor/RConn1 -- ua_afe/LConn1
  Current Sensor/RConn2 -- ua/RConn1
  Voltage Sensor1/RConn1 -- ub_afe/LConn1
  Voltage Sensor2/LConn1 -- Uc/RConn1 -- Current Sensor2/LConn1
  Current Sensor/LConn1 -- Ua/RConn1 -- Voltage Sensor/LConn1
  Current Sensor1/RConn2 -- ub/RConn1
  Voltage Sensor2/RConn1 -- uc_afe/LConn1
  ib_afe/LConn1 -- Current Sensor1/RConn1
  ia_afe/LConn1 -- Current Sensor/RConn1
  ic_afe/LConn1 -- Current Sensor2/RConn1
  Current Sensor2/RConn2 -- uc/RConn1

== system afe_inv_psm_param/afe_abc_inv_psm_mod1/LCL_filter/threephase_vi_measures_stack1 ==
  Bus Creator : BusCreator  Inputs=6
  Current Sensor : fl_lib/Electrical/Electrical Sensors/Current Sensor
  Current Sensor1 : fl_lib/Electrical/Electrical Sensors/Current Sensor
  Current Sensor2 : fl_lib/Electrical/Electrical Sensors/Current Sensor
  Electrical Reference1 : fl_lib/Electrical/Electrical Elements/Electrical Reference
  Gain1 : Gain  Gain=1/param.afe.hw.ubez
  Gain2 : Gain  Gain=1/param.afe.hw.ubez
  Gain3 : Gain  Gain=1/param.afe.hw.ubez
  Gain4 : Gain  Gain=1/param.afe.hw.ibez
  Gain5 : Gain  Gain=1/param.afe.hw.ibez
  Gain6 : Gain  Gain=1/param.afe.hw.ibez
  Selector : Selector  InputPortWidth=6  IndexOptions=Index vector (dialog)  Indices=[1 2 3]  OutputSizes=1  RuntimeRangeChecks=off
  Selector1 : Selector  InputPortWidth=6  IndexOptions=Index vector (dialog)  Indices=[4 5 6]  OutputSizes=1  RuntimeRangeChecks=off
  Voltage Sensor : fl_lib/Electrical/Electrical Sensors/Voltage Sensor
  Voltage Sensor1 : fl_lib/Electrical/Electrical Sensors/Voltage Sensor
  Voltage Sensor2 : fl_lib/Electrical/Electrical Sensors/Voltage Sensor
  ia_grid : nesl_utility/PS-Simulink Converter  PhysicalDomain=network_engine_domain  SubClassName=ps_output  LeftPortType=input  RightPortType=output  PseudoPeriodic=off  Frequencies=[]  VectorFormat=1-D array  Unit=A  AffineConversion=off
  ib_grid : nesl_utility/PS-Simulink Converter  PhysicalDomain=network_engine_domain  SubClassName=ps_output  LeftPortType=input  RightPortType=output  PseudoPeriodic=off  Frequencies=[]  VectorFormat=1-D array  Unit=A  AffineConversion=off
  ic_grid : nesl_utility/PS-Simulink Converter  PhysicalDomain=network_engine_domain  SubClassName=ps_output  LeftPortType=input  RightPortType=output  PseudoPeriodic=off  Frequencies=[]  VectorFormat=1-D array  Unit=A  AffineConversion=off
  ua_grid : nesl_utility/PS-Simulink Converter  PhysicalDomain=network_engine_domain  SubClassName=ps_output  LeftPortType=input  RightPortType=output  PseudoPeriodic=off  Frequencies=[]  VectorFormat=1-D array  Unit=V  AffineConversion=off
  ub_grid : nesl_utility/PS-Simulink Converter  PhysicalDomain=network_engine_domain  SubClassName=ps_output  LeftPortType=input  RightPortType=output  PseudoPeriodic=off  Frequencies=[]  VectorFormat=1-D array  Unit=V  AffineConversion=off
  uc_grid : nesl_utility/PS-Simulink Converter  PhysicalDomain=network_engine_domain  SubClassName=ps_output  LeftPortType=input  RightPortType=output  PseudoPeriodic=off  Frequencies=[]  VectorFormat=1-D array  Unit=V  AffineConversion=off
  Ua : PMIOPort  Side=Left
  ua : PMIOPort  Port=2  Side=Right
  Ub : PMIOPort  Port=3  Side=Left
  ub : PMIOPort  Port=4  Side=Right
  Uc : PMIOPort  Port=5  Side=Left
  uc : PMIOPort  Port=6  Side=Right
  tag scope: ig_abc_pu_mod1=global, ug_abc_pu_mod1=global
  wires:
  Selector1/1 -> [ig_abc_pu_mod1]
  uc_grid/1 -> Gain3/1
  ub_grid/1 -> Gain2/1
  ua_grid/1 -> Gain1/1
  ic_grid/1 -> Gain5/1
  ia_grid/1 -> Gain6/1
  ib_grid/1 -> Gain4/1
  Selector/1 -> [ug_abc_pu_mod1]
  Bus Creator/1 -> Selector1/1, Selector/1  "vi_data"
  Gain1/1 -> Bus Creator/1  "ua_grid_pu"
  Gain2/1 -> Bus Creator/2  "ub_grid_pu"
  Gain3/1 -> Bus Creator/3  "uc_grid_pu"
  Gain6/1 -> Bus Creator/4  "ia_grid_pu"
  Gain4/1 -> Bus Creator/5  "ib_grid_pu"
  Gain5/1 -> Bus Creator/6  "ic_grid_pu"
  connections:
  Current Sensor2/RConn2 -- uc/RConn1
  ic_grid/LConn1 -- Current Sensor2/RConn1
  ia_grid/LConn1 -- Current Sensor/RConn1
  ib_grid/LConn1 -- Current Sensor1/RConn1
  Voltage Sensor2/RConn1 -- uc_grid/LConn1
  Current Sensor1/RConn2 -- ub/RConn1
  Voltage Sensor/LConn1 -- Current Sensor/LConn1 -- Ua/RConn1
  Current Sensor2/LConn1 -- Voltage Sensor2/LConn1 -- Uc/RConn1
  Voltage Sensor1/RConn1 -- ub_grid/LConn1
  Current Sensor/RConn2 -- ua/RConn1
  Voltage Sensor/RConn1 -- ua_grid/LConn1
  Voltage Sensor1/RConn2 -- Voltage Sensor2/RConn2 -- Voltage Sensor/RConn2 -- Electrical Reference1/LConn1
  Voltage Sensor1/LConn1 -- Current Sensor1/LConn1 -- Ub/RConn1

== system afe_inv_psm_param/afe_abc_inv_psm_mod1/L_filter/threephase_vi_measures_stack ==
  Bus Creator : BusCreator  Inputs=6
  Current Sensor : fl_lib/Electrical/Electrical Sensors/Current Sensor
  Current Sensor1 : fl_lib/Electrical/Electrical Sensors/Current Sensor
  Current Sensor2 : fl_lib/Electrical/Electrical Sensors/Current Sensor
  Electrical Reference1 : fl_lib/Electrical/Electrical Elements/Electrical Reference
  Gain : Gain  Gain=1/param.psm.machine.ibez
  Gain1 : Gain  Gain=1/param.psm.machine.ibez
  Gain2 : Gain  Gain=1/param.psm.machine.ibez
  Gain3 : Gain  Gain=1/param.psm.machine.ubez
  Gain4 : Gain  Gain=1/param.psm.machine.ubez
  Gain5 : Gain  Gain=1/param.psm.machine.ubez
  Selector : Selector  InputPortWidth=6  IndexOptions=Index vector (dialog)  Indices=[1 2 3]  OutputSizes=1  RuntimeRangeChecks=off
  Selector1 : Selector  InputPortWidth=6  IndexOptions=Index vector (dialog)  Indices=[4 5 6]  OutputSizes=1  RuntimeRangeChecks=off
  Sum : Sum  Inputs=+++
  Voltage Sensor : fl_lib/Electrical/Electrical Sensors/Voltage Sensor
  Voltage Sensor1 : fl_lib/Electrical/Electrical Sensors/Voltage Sensor
  Voltage Sensor2 : fl_lib/Electrical/Electrical Sensors/Voltage Sensor
  iu_inv : nesl_utility/PS-Simulink Converter  PhysicalDomain=network_engine_domain  SubClassName=ps_output  LeftPortType=input  RightPortType=output  PseudoPeriodic=off  Frequencies=[]  VectorFormat=1-D array  Unit=A  AffineConversion=off
  iv_inv : nesl_utility/PS-Simulink Converter  PhysicalDomain=network_engine_domain  SubClassName=ps_output  LeftPortType=input  RightPortType=output  PseudoPeriodic=off  Frequencies=[]  VectorFormat=1-D array  Unit=A  AffineConversion=off
  iw_inv : nesl_utility/PS-Simulink Converter  PhysicalDomain=network_engine_domain  SubClassName=ps_output  LeftPortType=input  RightPortType=output  PseudoPeriodic=off  Frequencies=[]  VectorFormat=1-D array  Unit=A  AffineConversion=off
  uu_inv : nesl_utility/PS-Simulink Converter  PhysicalDomain=network_engine_domain  SubClassName=ps_output  LeftPortType=input  RightPortType=output  PseudoPeriodic=off  Frequencies=[]  VectorFormat=1-D array  Unit=V  AffineConversion=off
  uv_inv : nesl_utility/PS-Simulink Converter  PhysicalDomain=network_engine_domain  SubClassName=ps_output  LeftPortType=input  RightPortType=output  PseudoPeriodic=off  Frequencies=[]  VectorFormat=1-D array  Unit=V  AffineConversion=off
  uw_inv : nesl_utility/PS-Simulink Converter  PhysicalDomain=network_engine_domain  SubClassName=ps_output  LeftPortType=input  RightPortType=output  PseudoPeriodic=off  Frequencies=[]  VectorFormat=1-D array  Unit=V  AffineConversion=off
  Uu : PMIOPort  Side=Left
  uu : PMIOPort  Port=2  Side=Right
  Uv : PMIOPort  Port=3  Side=Left
  uv : PMIOPort  Port=4  Side=Right
  Uw : PMIOPort  Port=5  Side=Left
  uw : PMIOPort  Port=6  Side=Right
  tag scope: is_uvw_cm_mod1=global, is_uvw_pu_mod1=global, us_uvw_pu_mod1=global
  wires:
  Bus Creator/1 -> Selector/1, Selector1/1  "vi_data"
  Selector/1 -> [us_uvw_pu_mod1]
  iv_inv/1 -> Sum/2, Gain1/1  "iv_inv"
  iu_inv/1 -> Sum/1, Gain/1  "iu_inv"
  iw_inv/1 -> Sum/3, Gain2/1  "iw_inv"
  uu_inv/1 -> Gain3/1  "uu_inv"
  uv_inv/1 -> Gain4/1  "uv_inv"
  uw_inv/1 -> Gain5/1  "uw_inv"
  Selector1/1 -> [is_uvw_pu_mod1]
  Gain/1 -> Bus Creator/4  "iu_inv_pu"
  Gain1/1 -> Bus Creator/5  "iv_inv_pu"
  Gain2/1 -> Bus Creator/6  "iw_inv_pu"
  Gain3/1 -> Bus Creator/1  "uu_inv_pu"
  Gain4/1 -> Bus Creator/2  "uv_inv_pu"
  Gain5/1 -> Bus Creator/3  "uw_inv_pu"
  Sum/1 -> [is_uvw_cm_mod1]
  connections:
  Current Sensor1/LConn1 -- Uv/RConn1 -- Voltage Sensor1/LConn1
  Electrical Reference1/LConn1 -- Voltage Sensor/RConn2 -- Voltage Sensor2/RConn2 -- Voltage Sensor1/RConn2
  Voltage Sensor/RConn1 -- uu_inv/LConn1
  Current Sensor/RConn2 -- uu/RConn1
  Voltage Sensor1/RConn1 -- uv_inv/LConn1
  Voltage Sensor2/LConn1 -- Uw/RConn1 -- Current Sensor2/LConn1
  Current Sensor/LConn1 -- Uu/RConn1 -- Voltage Sensor/LConn1
  Current Sensor1/RConn2 -- uv/RConn1
  Voltage Sensor2/RConn1 -- uw_inv/LConn1
  iv_inv/LConn1 -- Current Sensor1/RConn1
  iu_inv/LConn1 -- Current Sensor/RConn1
  iw_inv/LConn1 -- Current Sensor2/RConn1
  Current Sensor2/RConn2 -- uw/RConn1

== system afe_inv_psm_param/afe_abc_inv_psm_mod1/afe/sv_pwm ==
  duties_uvw : Inport
  Bus Selector2 : BusSelector  OutputSignals=du(k),dv(k),dw(k)
  Constant1 : Constant  Value=param.afe.behav.pwm_phase_shift_mod1
  modulator1 : Subsystem
  td2tc_1 : TransferFcn  Denominator=[param.glb_time.tc 1]
  td2tc_2 : TransferFcn  Denominator=[param.glb_time.tc 1]
  td2tc_3 : TransferFcn  Denominator=[param.glb_time.tc 1]
  gate_cmds : Outport
  wires:
  modulator1/1(gate_cmds) -> gate_cmds/1
  Constant1/1 -> modulator1/4(phase)
  Bus Selector2/1 -> td2tc_1/1  "<du(k)>"
  Bus Selector2/2 -> td2tc_2/1  "<dv(k)>"
  Bus Selector2/3 -> td2tc_3/1  "<dw(k)>"
  duties_uvw/1 -> Bus Selector2/1
  td2tc_1/1 -> modulator1/1(u)  "du(t)"
  td2tc_3/1 -> modulator1/3(w)  "dw(t)"
  td2tc_2/1 -> modulator1/2(v)  "dv(t)"

== system afe_inv_psm_param/afe_abc_inv_psm_mod1/afe/three_phase_inverter_ideal_switch_based_model ==
  gate_commands : Inport
  three_phase_inverter_ideal_switch_based_model : three_phase_inverter_ideal_switch_based_model/three phase inverter ideal switch based model  Ron_ideal_switch=param.afe.ideal_switch.Rds_on  Vth=param.afe.ideal_switch.Vth  Vgamma=param.afe.ideal_switch.Vdon_diode  Rdon_diode=param.afe.ideal_switch.Rdon_diode  Csnubber=param.afe.ideal_switch.Csnubber  Rsnubber=param.afe.ideal_switch.Rsnubber
  udc(+) : PMIOPort  Side=Left
  u : PMIOPort  Port=2  Side=Right
  v : PMIOPort  Port=3  Side=Right
  udc(-) : PMIOPort  Port=4  Side=Left
  w : PMIOPort  Port=5  Side=Right
  wires:
  gate_commands/1 -> three_phase_inverter_ideal_switch_based_model/1
  connections:
  three_phase_inverter_ideal_switch_based_model/LConn1 -- udc(+)/RConn1
  three_phase_inverter_ideal_switch_based_model/RConn3 -- w/RConn1
  three_phase_inverter_ideal_switch_based_model/RConn2 -- v/RConn1
  three_phase_inverter_ideal_switch_based_model/LConn2 -- udc(-)/RConn1
  three_phase_inverter_ideal_switch_based_model/RConn1 -- u/RConn1
